simulink model "MPSFP4NFGA"  (R2026b)
settings: Solver=ode15s  MaxStep=1E-3
libraries: slpidlib x1
settings Model: LastModifiedBy=Neltzon Farid
settings DataIOCC: DSMLogging=off  ReturnWorkspaceOutputs=off  SaveOutput=off  SignalLogging=off  TimeSaveName=t
settings DebuggingCC: AlgebraicLoopMsg=none  ArtificialAlgebraicLoopMsg=none  MaxConsecutiveZCsMsg=none
settings SimscapeCC: SimscapeLogType=all  SimscapeNominalValues="[{\"value\":\"1\",\"unit\":\"A\"},{\"value\":\"1\",\"unit\":\"bar\"},{\"value\":\"1\",\"unit\":\"cm^2\"},{\"value\":\"1\",\"unit\":\"cm^3/s\"},{\"value\":\"1\",\"unit\":\"kJ/kg\"},{\"value\":\"1\",\"unit\":\"kW\"},{\"value\":\"1\",\"unit\":\"l\"},{\"value\":\"1\",\"unit\":\"N\"},{\"value\":\"1\",\"unit\":\"N*m\"},{\"value\":\"1\",\"unit\":\"V\"},{\"value\":\"0.001\",\"unit\":\"Wb\"}]"  SimscapeUseEnergyAccounting=off

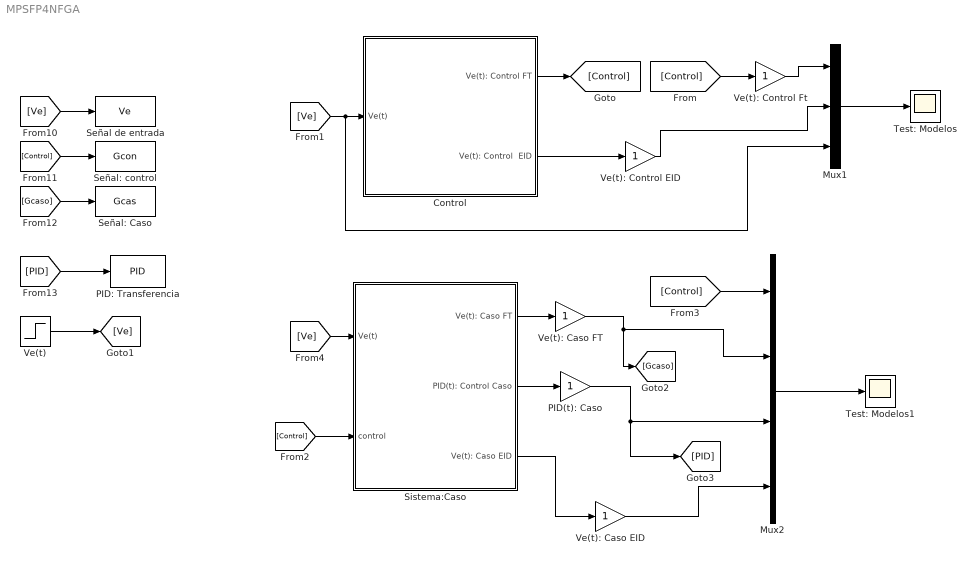
== system MPSFP4NFGA ==
  Control : Subsystem
  Mux1 : Mux  Inputs=3
  Mux2 : Mux
  PID(t): Caso : Gain
  PID: Transferencia : ToWorkspace  VariableName=PID  SampleTime=-1
  Señal de entrada : ToWorkspace  VariableName=Ve  SampleTime=-1
  Señal: Caso : ToWorkspace  VariableName=Gcas  SampleTime=-1
  Señal: control : ToWorkspace  VariableName=Gcon  SampleTime=-1
  Sistema:Caso : Subsystem
  Test: Modelos : Scope
      settings: ActiveDisplayYMinimum=-0.83442104468950684  ActiveDisplayYMaximum=1.7059795595996836  YLabel=V(t)
  Test: Modelos1 : Scope
      settings: ActiveDisplayYMinimum=-0.74389  ActiveDisplayYMaximum=1.2755  YLabel=V(t)
  Ve(t) : Step  Time=0  SampleTime=0
  Ve(t): Caso EID : Gain
  Ve(t): Caso FT : Gain
  Ve(t): Control EID : Gain
  Ve(t): Control Ft : Gain
  wires:
  Mux1/1 -> Test: Modelos/1
  [Ve] -> Mux1/3, Control/1(Ve(t))
  [Control] -> Señal: control/1
  [Gcaso] -> Señal: Caso/1
  [Ve] -> Señal de entrada/1
  [PID] -> PID: Transferencia/1
  Ve(t)/1 -> [Ve]
  [Control] -> Ve(t): Control Ft/1
  Sistema:Caso/2(PID(t): Control Caso) -> PID(t): Caso/1
  Mux2/1 -> Test: Modelos1/1
  [Control] -> Sistema:Caso/2(control)
  [Ve] -> Sistema:Caso/1(Ve(t))
  Sistema:Caso/1(Ve(t): Caso FT) -> Ve(t): Caso FT/1
  Ve(t): Caso FT/1 -> Mux2/2, [Gcaso]
  [Control] -> Mux2/1
  PID(t): Caso/1 -> [PID], Mux2/3
  Control/1(Ve(t): Control FT) -> [Control]
  Ve(t): Control Ft/1 -> Mux1/1
  Control/2(Ve(t): Control  EID) -> Ve(t): Control EID/1
  Ve(t): Control EID/1 -> Mux1/2
  Sistema:Caso/3(Ve(t): Caso EID) -> Ve(t): Caso EID/1
  Ve(t): Caso EID/1 -> Mux2/4

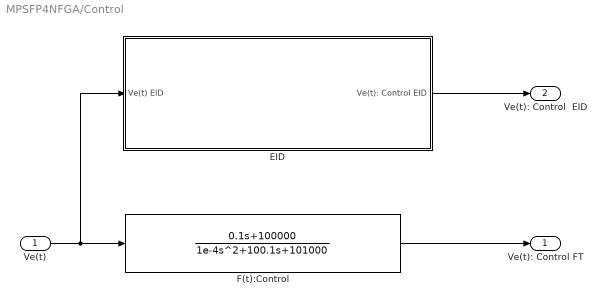
== system MPSFP4NFGA/Control ==
  Ve(t) : Inport
  EID : Subsystem
  F(t):Control : TransferFcn  Numerator=[0.1,100000]  Denominator=[1e-4,100.1,101000]
  Ve(t): Control FT : Outport
  Ve(t): Control  EID : Outport  Port=2
  wires:
  Ve(t)/1 -> EID/1(Ve(t) EID), F(t):Control/1
  F(t):Control/1 -> Ve(t): Control FT/1
  EID/1(Ve(t): Control EID) -> Ve(t): Control  EID/1

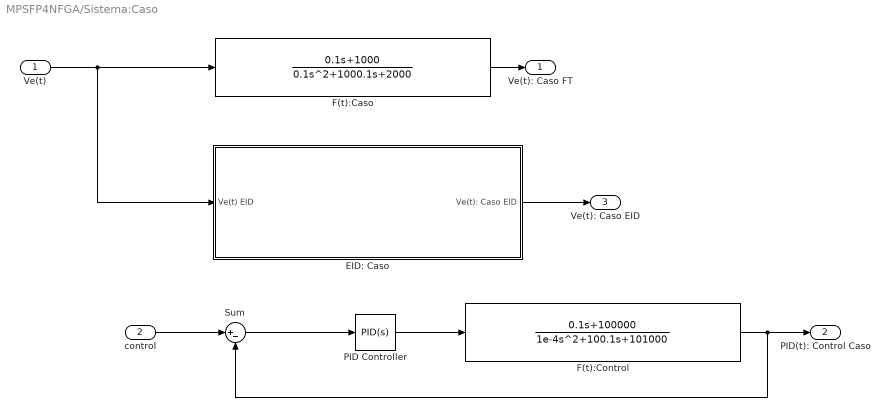
== system MPSFP4NFGA/Sistema:Caso ==
  Ve(t) : Inport
  control : Inport  Port=2
  EID: Caso : Subsystem
  F(t):Caso : TransferFcn  Numerator=[0.1,1000]  Denominator=[0.1,1000.1,2000]
  F(t):Control : TransferFcn  Numerator=[0.1,100000]  Denominator=[1e-4,100.1,101000]
  PID Controller : slpidlib/PID Controller  Controller=PID  Form=Parallel  TimeDomain=Continuous-time  UseExternalTs=off  SampleTime=-1  IntegratorMethod=Forward Euler  FilterMethod=Forward Euler  ControllerParametersSource=internal  P=9.36224920314089  I=30810.6473163972  UseKiTs=off  D=0.000285041688230155  UseExternalDerivativeSource=off  N=12954.4724615466  UseFilter=on  TunerSelectOption=Transfer Function Based (PID Tuner App)  InitialConditionSource=internal  InitialConditionForIntegrator=0  InitialConditionForFilter=0  DifferentiatorICPrevScaledInput=0  ExternalReset=none  TrackingMode=off  Kt=1  LimitOutput=off  SatLimitsSource=internal  UpperSaturationLimit=inf  LowerSaturationLimit=-inf  LinearizeAsGain=on  AntiWindupMode=none  Kb=1  LimitIntegrator=off  UpperIntegratorSaturationLimit=inf  LowerIntegratorSaturationLimit=-inf  POutMin=[]  POutMax=[]  IOutMin=[]  IOutMax=[]  DOutMin=[]  DOutMax=[]  NOutMin=[]  NOutMax=[]  SumOutMin=[]  SumOutMax=[]  SaturationOutMin=[]  SaturationOutMax=[]  PParamMin=[]  PParamMax=[]  IParamMin=[]  IParamMax=[]  DParamMin=[]  DParamMax=[]  NParamMin=[]  NParamMax=[]  KbParamMin=[]  KbParamMax=[]  KtParamMin=[]  KtParamMax=[]  KbOutMin=[]  KbOutMax=[]  KtOutMin=[]  KtOutMax=[]  IntegratorOutMin=[]  IntegratorOutMax=[]  FilterOutMin=[]  FilterOutMax=[]  SumI1OutMin=[]  SumI1OutMax=[]  SumI2OutMin=[]  SumI2OutMax=[]  SumI3OutMin=[]  SumI3OutMax=[]  SumI4OutMin=[]  SumI4OutMax=[]  SumDOutMin=[]  SumDOutMax=[]  DifferentiatorOutMin=[]  DifferentiatorOutMax=[]  FilterDiffOutCoefMin=[]  FilterDiffOutCoefMax=[]  ReciprocalOutMin=[]  ReciprocalOutMax=[]  SumDenOutMin=[]  SumDenOutMax=[]  SumNumOutMin=[]  SumNumOutMax=[]  DivideOutMin=[]  DivideOutMax=[]  UdiffTsProdOutMin=[]  UdiffTsProdOutMax=[]  NTsProdOutMin=[]  NTsProdOutMax=[]  UintegralTsProdOutMin=[]  UintegralTsProdOutMax=[]  UngainTsProdOutMin=[]  UngainTsProdOutMax=[]  ClampingZeroOutDataTypeStr=Inherit: Inherit via back propagation  ClampingZeroOutMin=[]  ClampingZeroOutMax=[]  FilterDenConstantOutDataTypeStr=Inherit: Inherit via back propagation  FilterDenConstantOutMin=[]  FilterDenConstantOutMax=[]  PCopyOutDataTypeStr=Inherit: Inherit via back propagation  PCopyOutMin=[]  PCopyOutMax=[]  NCopyOutDataTypeStr=Inherit: Inherit via back propagation  NCopyOutMin=[]  NCopyOutMax=[]  IntegratorContinuousStateAttributes=''  IntegratorStateMustResolveToSignalObject=off  IntegratorRTWStateStorageClass=Auto  FilterContinuousStateAttributes=''  FilterStateMustResolveToSignalObject=off  FilterRTWStateStorageClass=Auto  ParallelPVariant=InternalParameters  IdealPVariant=Disabled  IVariant=InternalParameters  DVariant=InternalParameters  IntegratorVariant=Continuous  SatVariant=Disabled  AWVariant=Passthrough  PCopyVariant=Disabled  TRVariant=Disabled  FdbkBlocksVariant=Forward  IdealPFdbkVariant=Disabled  SatFdbkVariant=Disabled  DerivativeFilterVariant=ContFilter  NVariant=InternalParameters  NCopyVariant=Disabled  FilterICVariant=InternalICsFilter  IntegratorICVariant=InternalICs  ExternalResetVariant=Disabled  TRSumVariant=Passthrough  SumFdbkVariant=Disabled  SumVariant=Sum_PID  TsampFilterVariant=InternalTs  TsampNgainVariant=Passthrough  TsampIntegralVariant=Disabled_SignalSpec  ExternalSaturationOutDataTypeStr=Inherit: Same as second input  DerivativeSourceVariant=ErrorSignal  PreIntVariant=InternalPreInt
  Sum : Sum  Inputs=|+-
  Ve(t): Caso FT : Outport
  PID(t): Control Caso : Outport  Port=2
  Ve(t): Caso EID : Outport  Port=3
  wires:
  Ve(t)/1 -> EID: Caso/1(Ve(t) EID), F(t):Caso/1
  F(t):Caso/1 -> Ve(t): Caso FT/1
  F(t):Control/1 -> Sum/2, PID(t): Control Caso/1
  PID Controller/1 -> F(t):Control/1
  Sum/1 -> PID Controller/1
  control/1 -> Sum/1
  EID: Caso/1(Ve(t): Caso EID) -> Ve(t): Caso EID/1

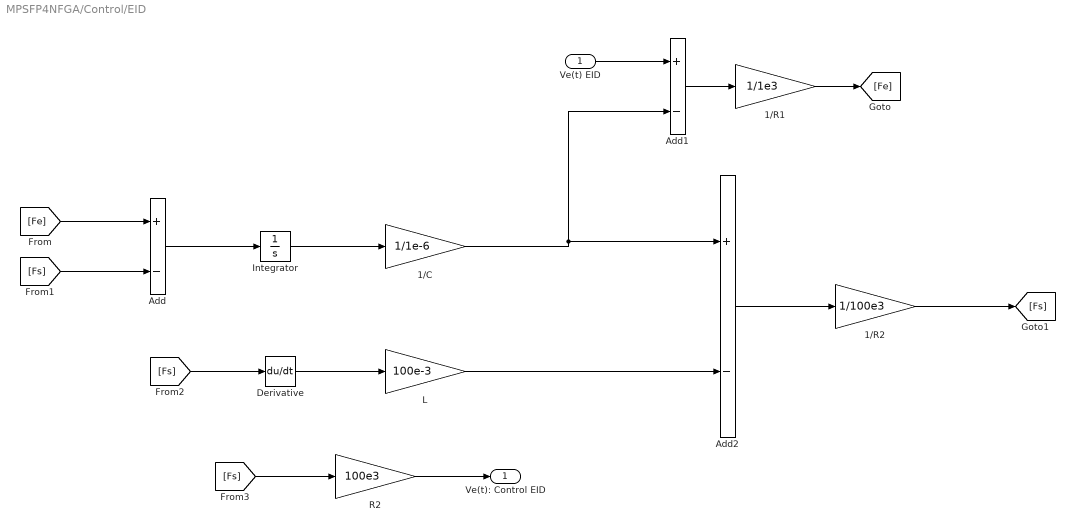
== system MPSFP4NFGA/Control/EID ==
  Ve(t) EID : Inport
  1/C : Gain  Gain=1/1e-6
  1/R1 : Gain  Gain=1/1e3
  1/R2 : Gain  Gain=1/100e3
  Add : Sum  Inputs=+-
  Add1 : Sum  Inputs=+-
  Add2 : Sum  Inputs=+-
  Derivative : Derivative
  Integrator : Integrator
  L : Gain  Gain=100e-3
  R2 : Gain  Gain=100e3
  Ve(t): Control EID : Outport
  wires:
  R2/1 -> Ve(t): Control EID/1
  Add1/1 -> 1/R1/1
  [Fe] -> Add/1
  [Fs] -> Derivative/1
  1/C/1 -> Add2/1, Add1/2
  1/R2/1 -> [Fs]
  Add2/1 -> 1/R2/1
  Derivative/1 -> L/1
  Integrator/1 -> 1/C/1
  [Fs] -> R2/1
  1/R1/1 -> [Fe]
  Ve(t) EID/1 -> Add1/1
  L/1 -> Add2/2
  [Fs] -> Add/2
  Add/1 -> Integrator/1

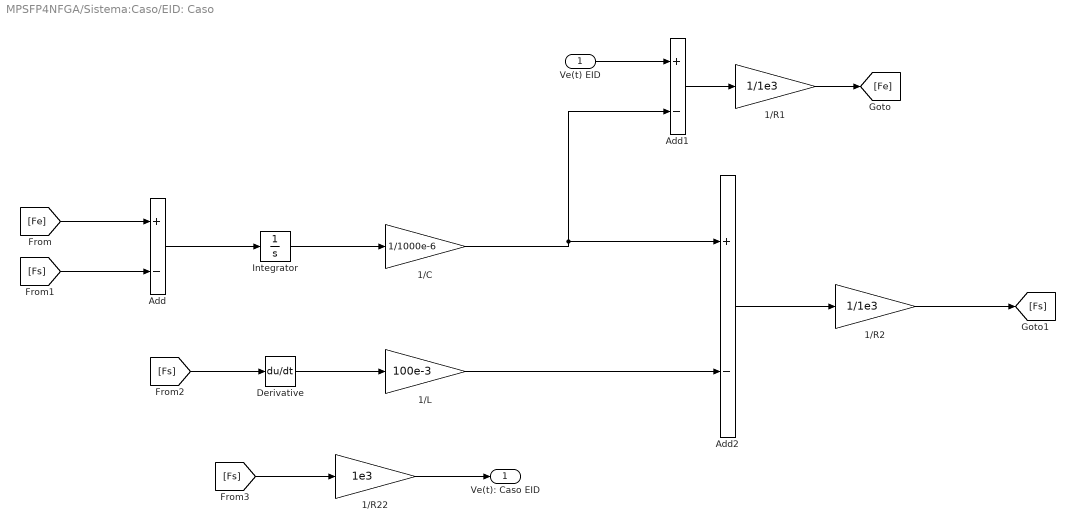
== system MPSFP4NFGA/Sistema:Caso/EID: Caso ==
  Ve(t) EID : Inport
  1/C : Gain  Gain=1/1000e-6
  1/L : Gain  Gain=100e-3
  1/R1 : Gain  Gain=1/1e3
  1/R2 : Gain  Gain=1/1e3
  1/R22 : Gain  Gain=1e3
  Add : Sum  Inputs=+-
  Add1 : Sum  Inputs=+-
  Add2 : Sum  Inputs=+-
  Derivative : Derivative
  Integrator : Integrator
  Ve(t): Caso EID : Outport
  wires:
  1/R22/1 -> Ve(t): Caso EID/1
  Add1/1 -> 1/R1/1
  [Fe] -> Add/1
  [Fs] -> Derivative/1
  1/C/1 -> Add2/1, Add1/2
  1/R2/1 -> [Fs]
  Add2/1 -> 1/R2/1
  Derivative/1 -> 1/L/1
  Integrator/1 -> 1/C/1
  [Fs] -> 1/R22/1
  1/R1/1 -> [Fe]
  Ve(t) EID/1 -> Add1/1
  1/L/1 -> Add2/2
  [Fs] -> Add/2
  Add/1 -> Integrator/1
